simulink model "ASM_Traffic_new"  (R2024a)
settings: Solver=ode1  StartTime=SIM.tstart.v  StopTime=SIM.tend.v  FixedStep=SIM.StepSize.v  RelTol=1e-3
PostLoadFcn:
  | if any(exist('dsrtsu_mdlpostloadfcn', 'file') ~= 0), dsrtsu_mdlpostloadfcn('Execute', bdroot); end
  | try, asm_mdl_postloadfcn(bdroot, 'UpdateModel', 3600); catch, disp(lasterr); end,
InitFcn:
  | , if any(exist('rtifpga_mdlclblib', 'file') ~= 0), rtifpga_mdlclblib('Init', bdroot); end,
  | , if any(exist('dsmpb_private', 'file') ~= 0), dsmpb_private('dsmpb_mdlclblib', 'Init', bdroot); end,
undefined symbols (not defined in the file): _to_, a0b2, ASM_BrakeHydraulics_DemoSystems, ASM_VehicleDynamics_DemoSystems, b98103fe8ad365046cd0, BrakeCircuit, CPT, Crankshaft, DiscIntNeverNeededParam, dsmsi, FinalDriveAssembly, MDL, ModeSignals, Pos_BrakePedal_Maneuver, rad, RefSignals, s_to_rpm, SIM, SoftECU, Suspension, Tire, Transmission
libraries: ASM_Traffic_lib x135, simulink x100, ASM_Utils_lib x77, ASM_VehicleDynamics_lib x70, ASM_Environment_lib x22, dsmpblib x20, dsmsilib x15, MDLD_Utils_lib x10, ASM_BrakeHydraulics_lib x3
(part 3 of 63)

== system ASM_Traffic_new/AnimationInterface/Vehicle_Lights ==
  VehicleDynamics_Animation : Inport
  Environment_Animation : Inport  Port=2
  Bus Selector : BusSelector  OutputSignals=Sw_ManualControl_Lights[1Maneuver|2Manual],Sw_BrakeLight[0Off|1On],Sw_TurnLights[0Off|1Left|2Right|3Both],ASM_Vehicle_TurnLights[]
  Bus Selector13 : BusSelector  OutputSignals=p_Brake[FL;FR;RL;RR][bar]
  Cmp_BrakePres : simulink/Logic and Bit Operations/Compare To Constant  relop=>  const=3  OutDataTypeStr=boolean
  Coding : Subsystem
  Compare_Hazard : simulink/Logic and Bit Operations/Compare To Constant  relop===  const=3  OutDataTypeStr=boolean
  Compare_Turnlight_L : simulink/Logic and Bit Operations/Compare To Constant  relop===  const=1.0  OutDataTypeStr=boolean
  Compare_Turnlight_R : simulink/Logic and Bit Operations/Compare To Constant  relop===  const=2  OutDataTypeStr=boolean
  Data Type Conversion1 : DataTypeConversion  OutDataTypeStr=boolean  SaturateOnIntegerOverflow=off  RndMeth=Floor
  Data Type Conversion2 : DataTypeConversion  OutDataTypeStr=uint32  SaturateOnIntegerOverflow=off  RndMeth=Floor
  Data Type Conversion3 : DataTypeConversion  OutDataTypeStr=uint32  SaturateOnIntegerOverflow=off  RndMeth=Floor
  Data Type Conversion4 : DataTypeConversion  OutDataTypeStr=uint32  SaturateOnIntegerOverflow=off  RndMeth=Floor
  Gain : Gain  Gain=1/4
  Multiport Switch : MultiPortSwitch  Inputs=2  SaturateOnIntegerOverflow=off  InputSameDT=off
  Multiport Switch4 : MultiPortSwitch  Inputs=2  SaturateOnIntegerOverflow=off  InputSameDT=off
  Mux : Mux  Inputs=3
  OR : Logic  Operator=OR  IconShape=distinctive  AllPortsSameDT=off  OutDataTypeStr=boolean
  OR1 : Logic  Operator=OR  IconShape=distinctive  AllPortsSameDT=off  OutDataTypeStr=boolean
  Sum of Elements : Sum  Inputs=+
  ASM_Vehicle_Lights : Outport  VectorParamsAs1DForOutWhenUnconnected=off
  wires:
  Bus Selector13/1 -> Sum of Elements/1  "<p_Brake[FL;FR;RL;RR][bar]>"
  Compare_Turnlight_L/1 -> OR/1
  Gain/1 -> Cmp_BrakePres/1
  Multiport Switch/1 -> Mux/1
  Data Type Conversion3/1 -> Multiport Switch/1, Multiport Switch4/1
  Compare_Hazard/1 -> OR/2, OR1/2
  Bus Selector/1 -> Data Type Conversion3/1  "<Sw_ManualControl_Lights[1Maneuver|2Manual]>"
  Bus Selector/3 -> Data Type Conversion2/1  "<Sw_TurnLights[0Off|1Left|2Right|3Both]>"
  Data Type Conversion4/1 -> Multiport Switch4/2
  Sum of Elements/1 -> Gain/1
  Bus Selector/4 -> Data Type Conversion4/1  "<ASM_Vehicle_TurnLights[]>"
  Bus Selector/2 -> Data Type Conversion1/1  "<Sw_BrakeLight[0Off|1On]>"
  Compare_Turnlight_R/1 -> OR1/1
  OR1/1 -> Mux/3
  Cmp_BrakePres/1 -> Multiport Switch/2
  Data Type Conversion2/1 -> Multiport Switch4/3
  OR/1 -> Mux/2
  Data Type Conversion1/1 -> Multiport Switch/3
  Multiport Switch4/1 -> Compare_Hazard/1, Compare_Turnlight_R/1, Compare_Turnlight_L/1
  Mux/1 -> Coding/1(In)
  Coding/1(Out) -> ASM_Vehicle_Lights/1
  Environment_Animation/1 -> Bus Selector/1
  VehicleDynamics_Animation/1 -> Bus Selector13/1

== system ASM_Traffic_new/DomainControl/DriverAssistance ==
  note: Driver Assistance
  In : Inport
  Control : Subsystem
  Interface_In : Subsystem
  Interface_Out : Subsystem
  SignalInterface : Subsystem
  Out : Outport  VectorParamsAs1DForOutWhenUnconnected=off
  wires:
  In/1 -> Interface_In/1(In)
  Interface_In/1(Out) -> SignalInterface/1(In), Control/1(Interface_In)
  Interface_Out/1(Out) -> Out/1
  Control/1(Control) -> Interface_Out/1(In)

== system ASM_Traffic_new/DomainControl/StartSystem ==
  note: Start System
  In : Inport
  Control : Subsystem
  Interface_In : Subsystem
  Interface_Out : Subsystem
  SignalInterface : Subsystem
  Out : Outport  VectorParamsAs1DForOutWhenUnconnected=off
  wires:
  In/1 -> Interface_In/1(In)
  Interface_In/1(Out) -> SignalInterface/1(In), Control/1(Interface_In)
  Interface_Out/1(Out) -> Out/1
  Control/1(Control) -> Interface_Out/1(In)

== system ASM_Traffic_new/DomainControl/TorqueManager ==
  note: Torque Manager Basic
  In : Inport
  Control : Subsystem
  Interface_In : Subsystem
  Interface_Out : Subsystem
  SignalInterface : Subsystem
  Out : Outport  VectorParamsAs1DForOutWhenUnconnected=off
  wires:
  In/1 -> Interface_In/1(In)
  Control/1(Control) -> Interface_Out/1(In)
  Interface_In/1(Out) -> SignalInterface/1(In), Control/1(Interface_In)
  Interface_Out/1(Out) -> Out/1

== system ASM_Traffic_new/Driver/Interface_In ==
  note: Driver
  In : Inport
  Bus Creator1 : BusCreator  Inputs=1
  Bus Selector4 : BusSelector  OutputSignals=Environment.Plant.Sw_ModelPortBlocks[0Disabled|1Enabled],Environment.Plant.Sw_ModelDeskPlottingInterface[0Disabled|1Enabled],VehicleDynamics.Plant.v_x_Vehicle_CoG[km|h],VehicleDynamics.Plant.v_y_Vehicle_CoG[km|h],VehicleDynamics.Plant.Pos_x_Vehicle_CoorSys_E[m],VehicleDynamics.Plant.Pos_y_Vehicle_CoorSys_E[m],VehicleDynamics.Plant.Angle_Yaw_Vehicle_CoorSys_E[deg],VehicleDynamics.Plant.YawRate_Vehicle_CoG[deg|s],VehicleDynamics.Plant.m_TotalVehicle[kg],VehicleDynamics.Plant.F_Driving_Res[N],VehicleDynamics.Plant.Pos_x_CoG_Vehicle_Total[m],VehicleDynamics.Plant.Inertia_z_Vehicle_Total[kgm2],VehicleDynamics.Plant.CorneringStiffness_Tire_Front[N|rad],VehicleDynamics.Plant.CorneringStiffness_Tire_Rear[N|rad],VehicleDynamics.Plant.i_Steering_Mean[],Drivetrain.Plant.n_Engine[rpm],Drivetrain.Plant.omega_Out_Trm[rad|s],DomainControl.TorqueManager.Control.State_Engine[0|1|2|3|4],Environment.Plant.Reset_States[0|1],Environment.Plant.s_Vehicle_Init[m],Environment.Plant.Route_Direction_Init[],Environment.Plant.s_Total_Vehicle_Road[m],Environment.Plant.Curv_Preview_Road[1|m],Environment.Plant.Speed_Limit_Preview_Road[km|h],Environment.Plant.Pos_z_Preview_Road[m],Environment.Plant.Roll_Preview_Road[deg],Environment.Plant.Pitch_Preview_Road[deg],Environment.Plant.x_Preview_DriverCurv[m],Environment.Plant.y_Preview_DriverCurv[m],Environment.Plant.Pos_x_Preview_Road[m],Environment.Plant.Pos_y_Preview_Road[m],Environment.Plant.Dist_Border_Left[m],Environment.Plant.Dist_Border_Right[m],Environment.Plant.Curv_Vehicle_Road[1|m],Environment.Plant.Angle_Yaw_Veh_Road[deg],Environment.Plant.Pos_AccPedal_Maneuver[%],Environment.Plant.Pos_BrakePedal_Maneuver[%],Environment.Plant.Pos_ClutchPedal_Maneuver[%],Environment.Plant.Gear_Maneuver[],Environment.Plant.Angle_SteeringWheel_Maneuver[deg],Environment.Plant.SelectorLever_Maneuver[-3T|-2P|-1R|0N|1D],Environment.Plant.v_Vehicle_Ref_Maneuver[m|s],Environment.Plant.v_Vehicle_Preview_Ref_Maneuver[m|s],Environment.Plant.a_x_Max[m|s2],Environment.Plant.a_x_Min[m|s2],Environment.Plant.a_y_Max[m|s2],Environment.Plant.Gear_Max[0Off|1_n],Environment.Plant.a_x_Vehicle_Ref_TrafficDriver[m|s2],Environment.Plant.Width_Deadzone_LatCtrl[m],Environment.Plant.Pos_x_Ref_Vehicle_Road[m],Environment.Plant.Pos_y_Ref_Vehicle_Road[m],Environment.Plant.Enable_v_Init[0|1],Drivetrain.Plant.Mode_Transmission[1Manual|2Automatic],Environment.Plant.Mode_AcceleratorBrake[1Stim|2Driver],Environment.Plant.Mode_GearClutch[1Stim|2Driver|3OpenClutch|4RefGear],Environment.Plant.Mode_Steer[1Stim|2Driver|3Fix],Environment.Plant.Sw_LatDriver[1LatCtrl1|2LatCtrl2],Environment.Plant.Mode_LatCtrl[1Pos|2Yaw],Environment.Plant.Mode_AdaptVelocityToRoad[1Off|2On],Environment.Plant.Mode_ForceToRoad[1Off|2On],Environment.Plant.Mode_SelectorLever[1Stim|2Driver],Environment.Plant.Mode_CurvatureCalculation[1Road|2Driver],Environment.Plant.Mode_TrafficDriver[1Off|2On],Engine.Control.State_StartStop[1Off|2NotReady|3Ready|4EngStopped],Engine.Control.n_Engine_Idle_Set[rpm],Environment.Plant.Lane_ID_Vehicle[]
  ModelSignals : Subsystem
  Out : Outport  VectorParamsAs1DForOutWhenUnconnected=off
  wires:
  Bus Selector4/2 -> ModelSignals/2(Sw_ModelDeskPlottingInterface[0Disabled|1Enabled])  "<Sw_ModelDeskPlottingInterface[0Disabled|1Enabled]>"
  Bus Selector4/1 -> ModelSignals/1(Sw_ModelPortBlocks[0Disabled|1Enabled])  "<Sw_ModelPortBlocks[0Disabled|1Enabled]>"
  In/1 -> Bus Selector4/1
  Bus Selector4/51 -> ModelSignals/51(Pos_y_Ref_Vehicle_Road[m])  "<Pos_y_Ref_Vehicle_Road[m]>"
  Bus Selector4/50 -> ModelSignals/50(Pos_x_Ref_Vehicle_Road[m])  "<Pos_x_Ref_Vehicle_Road[m]>"
  Bus Selector4/49 -> ModelSignals/49(Width_Deadzone_LatCtrl[m])  "<Width_Deadzone_LatCtrl[m]>"
  Bus Selector4/48 -> ModelSignals/48(a_x_Vehicle_Ref_TrafficDriver[m|s2])  "<a_x_Vehicle_Ref_TrafficDriver[m|s2]>"
  Bus Selector4/47 -> ModelSignals/47(Gear_Max[0Off|1_n])  "<Gear_Max[0Off|1_n]>"
  Bus Selector4/46 -> ModelSignals/46(a_y_Max[m|s2])  "<a_y_Max[m|s2]>"
  Bus Selector4/45 -> ModelSignals/45(a_x_Min[m|s2])  "<a_x_Min[m|s2]>"
  Bus Selector4/44 -> ModelSignals/44(a_x_Max[m|s2])  "<a_x_Max[m|s2]>"
  Bus Selector4/43 -> ModelSignals/43(v_Vehicle_Preview_Ref_Maneuver[m|s])  "<v_Vehicle_Preview_Ref_Maneuver[m|s]>"
  Bus Selector4/42 -> ModelSignals/42(v_Vehicle_Ref_Maneuver[m|s])  "<v_Vehicle_Ref_Maneuver[m|s]>"
  Bus Selector4/41 -> ModelSignals/41(SelectorLever_Maneuver[-3T|-2P|-1R|0N|1D])  "<SelectorLever_Maneuver[-3T|-2P|-1R|0N|1D]>"
  Bus Selector4/40 -> ModelSignals/40(Angle_SteeringWheel_Maneuver[deg])  "<Angle_SteeringWheel_Maneuver[deg]>"
  Bus Selector4/39 -> ModelSignals/39(Gear_Maneuver[])  "<Gear_Maneuver[]>"
  Bus Selector4/38 -> ModelSignals/38(Pos_ClutchPedal_Maneuver[%])  "<Pos_ClutchPedal_Maneuver[%]>"
  Bus Selector4/37 -> ModelSignals/37(Pos_BrakePedal_Maneuver[%])  "<Pos_BrakePedal_Maneuver[%]>"
  Bus Selector4/36 -> ModelSignals/36(Pos_AccPedal_Maneuver[%])  "<Pos_AccPedal_Maneuver[%]>"
  Bus Selector4/35 -> ModelSignals/35(Angle_Yaw_Veh_Road[deg])  "<Angle_Yaw_Veh_Road[deg]>"
  Bus Selector4/34 -> ModelSignals/34(Curv_Veh_Road[1|m])  "<Curv_Vehicle_Road[1|m]>"
  Bus Selector4/33 -> ModelSignals/33(Dist_Border_Right[m])  "<Dist_Border_Right[m]>"
  Bus Selector4/32 -> ModelSignals/32(Dist_Border_Left[m])  "<Dist_Border_Left[m]>"
  Bus Selector4/31 -> ModelSignals/31(Pos_y_Preview_Road[m])  "<Pos_y_Preview_Road[m]>"
  Bus Selector4/30 -> ModelSignals/30(Pos_x_Preview_Road[m])  "<Pos_x_Preview_Road[m]>"
  Bus Selector4/29 -> ModelSignals/29(Pos_y_Preview_DriverCurv[m])  "<y_Preview_DriverCurv[m]>"
  Bus Selector4/28 -> ModelSignals/28(Pos_x_Preview_DriverCurv[m])  "<x_Preview_DriverCurv[m]>"
  Bus Selector4/27 -> ModelSignals/27(Pitch_Preview_Road[deg])  "<Pitch_Preview_Road[deg]>"
  Bus Selector4/26 -> ModelSignals/26(Roll_Preview_Road[deg])  "<Roll_Preview_Road[deg]>"
  Bus Selector4/25 -> ModelSignals/25(Pos_z_Preview_Road[m])  "<Pos_z_Preview_Road[m]>"
  Bus Selector4/24 -> ModelSignals/24(Speed_Limit_Preview_Road[km|h])  "<Speed_Limit_Preview_Road[km|h]>"
  Bus Selector4/23 -> ModelSignals/23(Curv_Preview_Road[1|m])  "<Curv_Preview_Road[1|m]>"
  Bus Selector4/22 -> ModelSignals/22(s_Total_Vehicle_Road[m])  "<s_Total_Vehicle_Road[m]>"
  Bus Selector4/21 -> ModelSignals/21(Route_Direction_Init[])  "<Route_Direction_Init[]>"
  Bus Selector4/20 -> ModelSignals/20(s_Vehicle_Init[m])  "<s_Vehicle_Init[m]>"
  Bus Selector4/19 -> ModelSignals/19(Reset_States[0|1])  "<Reset_States[0|1]>"
  Bus Creator1/1 -> Out/1
  Bus Selector4/52 -> ModelSignals/52(Enable_v_Init[0|1])  "<Enable_v_Init[0|1]>"
  Bus Selector4/53 -> ModelSignals/53(Mode_Transmission[1Manual|2Automatic])  "<Mode_Transmission[1Manual|2Automatic]>"
  Bus Selector4/54 -> ModelSignals/54(Mode_AcceleratorBrake[1Stim|2Driver])  "<Mode_AcceleratorBrake[1Stim|2Driver]>"
  Bus Selector4/55 -> ModelSignals/55(Mode_GearClutch[1Stim|2Driver|3OpenClutch|4RefGear])  "<Mode_GearClutch[1Stim|2Driver|3OpenClutch|4RefGear]>"
  Bus Selector4/56 -> ModelSignals/56(Mode_Steer[1Stim|2Driver|3Fix])  "<Mode_Steer[1Stim|2Driver|3Fix]>"
  Bus Selector4/57 -> ModelSignals/57(Sw_LatDriver[1LatCtrl1|2LatCtrl2])  "<Sw_LatDriver[1LatCtrl1|2LatCtrl2]>"
  Bus Selector4/58 -> ModelSignals/58(Mode_LatCtrl[1Pos|2Yaw])  "<Mode_LatCtrl[1Pos|2Yaw]>"
  Bus Selector4/59 -> ModelSignals/59(Mode_AdaptVelocityToRoad[1Off|2On])  "<Mode_AdaptVelocityToRoad[1Off|2On]>"
  Bus Selector4/60 -> ModelSignals/60(Mode_ForceToRoad[1Off|2On])  "<Mode_ForceToRoad[1Off|2On]>"
  Bus Selector4/61 -> ModelSignals/61(Mode_SelectorLever[1Stim|2Driver])  "<Mode_SelectorLever[1Stim|2Driver]>"
  Bus Selector4/62 -> ModelSignals/62(Mode_CurvatureCalculation[1Road|2Driver])  "<Mode_CurvatureCalculation[1Road|2Driver]>"
  Bus Selector4/63 -> ModelSignals/63(Mode_TrafficDriver[1Off|2On])  "<Mode_TrafficDriver[1Off|2On]>"
  Bus Selector4/65 -> ModelSignals/65(n_Engine_Idle_Set[rpm])  "<n_Engine_Idle_Set[rpm]>"
  Bus Selector4/64 -> ModelSignals/64(State_StartStop[1Off|2NotReady|3Ready|4EngStopped])  "<State_StartStop[1Off|2NotReady|3Ready|4EngStopped]>"
  Bus Selector4/18 -> ModelSignals/18(State_Engine[0|1|2|3|4])  "<State_Engine[0|1|2|3|4]>"
  Bus Selector4/17 -> ModelSignals/17(omega_Out_Trm[rad|s])  "<omega_Out_Trm[rad|s]>"
  Bus Selector4/16 -> ModelSignals/16(n_Engine[rpm])  "<n_Engine[rpm]>"
  Bus Selector4/15 -> ModelSignals/15(i_Steering_Mean[])  "<i_Steering_Mean[]>"
  Bus Selector4/14 -> ModelSignals/14(CorneringStiffness_Tire_Rear[N|rad])  "<CorneringStiffness_Tire_Rear[N|rad]>"
  Bus Selector4/13 -> ModelSignals/13(CorneringStiffness_Tire_Front[N|rad])  "<CorneringStiffness_Tire_Front[N|rad]>"
  Bus Selector4/12 -> ModelSignals/12(Inertia_z_Vehicle_Total[kgm2])  "<Inertia_z_Vehicle_Total[kgm2]>"
  Bus Selector4/11 -> ModelSignals/11(Pos_x_CoG_Vehicle_Total[m])  "<Pos_x_CoG_Vehicle_Total[m]>"
  Bus Selector4/10 -> ModelSignals/10(F_Driving_Res[N])  "<F_Driving_Res[N]>"
  Bus Selector4/9 -> ModelSignals/9(m_Total_Vehicle[kg])  "<m_TotalVehicle[kg]>"
  Bus Selector4/8 -> ModelSignals/8(YawRate_Vehicle[deg|s])  "<YawRate_Vehicle_CoG[deg|s]>"
  Bus Selector4/7 -> ModelSignals/7(Angle_Yaw_Vehicle_CoorSys_E[deg])  "<Angle_Yaw_Vehicle_CoorSys_E[deg]>"
  Bus Selector4/6 -> ModelSignals/6(Pos_y_Vehicle_CoorSys_E[m])  "<Pos_y_Vehicle_CoorSys_E[m]>"
  Bus Selector4/5 -> ModelSignals/5(Pos_x_Vehicle_CoorSys_E[m])  "<Pos_x_Vehicle_CoorSys_E[m]>"
  Bus Selector4/4 -> ModelSignals/4(v_y_Vehicle_CoG[km|h])  "<v_y_Vehicle_CoG[km|h]>"
  Bus Selector4/3 -> ModelSignals/3(v_x_Vehicle_CoG[km|h])  "<v_x_Vehicle_CoG[km|h]>"
  ModelSignals/1(Out) -> Bus Creator1/1
  Bus Selector4/66 -> ModelSignals/66(Lane_ID_Vehicle[])  "<Lane_ID_Vehicle[]>"

== system ASM_Traffic_new/Driver/Interface_Out ==
  note: Driver
  In : Inport
  Bus Creator1 : BusCreator  Inputs=1
  Bus Selector2 : BusSelector  OutputSignals=OutputSignals.Pos_AccPedal[%],OutputSignals.Pos_BrakePedal[%],OutputSignals.Pos_ClutchPedal[%],OutputSignals.Gear[],OutputSignals.SelectorLever[-3T|-2P|-1R|0N|1D],OutputSignals.s_Preview[m],OutputSignals.Angle_SteeringWheel[deg],LongitudinalController.LongCtrl.t_Preview[s]
  Plant_ModelSignals : Subsystem
  Out : Outport  VectorParamsAs1DForOutWhenUnconnected=off
  wires:
  Bus Selector2/6 -> Plant_ModelSignals/6(s_Preview[m])  "<s_Preview[m]>"
  Bus Selector2/8 -> Plant_ModelSignals/8(t_Preview_vRef_Driver[s])  "<t_Preview[s]>"
  Bus Selector2/5 -> Plant_ModelSignals/5(SelectorLever[-3T|-2P|-1R|0N|1D])  "<SelectorLever[-3T|-2P|-1R|0N|1D]>"
  Bus Selector2/4 -> Plant_ModelSignals/4(Gear[])  "<Gear[]>"
  Bus Selector2/3 -> Plant_ModelSignals/3(Pos_ClutchPedal[%])  "<Pos_ClutchPedal[%]>"
  Bus Selector2/2 -> Plant_ModelSignals/2(Pos_BrakePedal[%])  "<Pos_BrakePedal[%]>"
  Bus Selector2/1 -> Plant_ModelSignals/1(Pos_AccPedal[%])  "<Pos_AccPedal[%]>"
  In/1 -> Bus Selector2/1
  Bus Selector2/7 -> Plant_ModelSignals/7(Angle_SteeringWheel[deg])  "<Angle_SteeringWheel[deg]>"
  Bus Creator1/1 -> Out/1  "Driver"
  Plant_ModelSignals/1(Out) -> Bus Creator1/1

== system ASM_Traffic_new/Driver/Plant ==
  note: Driver
  Interface_In : Inport
  Driver : Subsystem
  UserInterface : Subsystem
  Plant : Outport  VectorParamsAs1DForOutWhenUnconnected=off
  wires:
  Driver/1(ASMSignalBus) -> Plant/1, UserInterface/1(In)
  Interface_In/1 -> Driver/2(Interface_In), UserInterface/2(Interface_In)
  UserInterface/1(Out) -> Driver/1(UserInterface)

== system ASM_Traffic_new/Driver/SignalInterface ==
  In : Inport
  ASMSignalInterface : Subsystem  mask(ASM_SIGNAL_INTERFACE){LabelTextfield=Driver}
      mask prompts: LabelTextfield "Label"
      mask help:
      | The ASMSignalInterface block processes the ASMSignalBus and provides a vector-based interface for each signal (e.g. ModelDesk Plotting).
      |
      | Always push the update button after you have changed the signal bus structure in order to synchronize the signal interface. The update may take a few seconds.
      | A modified model must be reloaded in ModelDesk to keep consistency of ModelDesk and simulation model plot signals. Therefore select ''Update Model'' from the ''Simulation Model'' context menu of the ModelDesk Project Navigator.
      settings: AttributesFormatString=Label: %<LabelTextfield>
      settings: CopyFcn=|
      | try
      |  set_param(gcb,'LinkStatus', 'none')
      | catch
      | end
      mask Help: eval(['asm_modelhelp(gcbh,''tool'',''ASM_Utils_lib'', ''ASMSIGNALINTERFACE'')'])
      mask DialogControl Hint Prompt: For changes of Label first apply change and then push "Update".
      mask DialogControl UpdateButton Prompt: Update
      mask DialogControl UpdateButton Callback: asm_mdld_plot_block_update(bdroot(gcb), 'update', 'current');
      mask DialogControl UpdateAllButton Prompt: Update All
      mask DialogControl UpdateAllButton Callback: asm_mdld_plot_block_update(bdroot(gcb), 'update', 'all');
  Bus Selector Disable Signals : BusSelector  OutputSignals=ExternalModel.Sw_ModelPortBlocks[0Disabled|1Enabled],ExternalModel.Sw_ModelDeskPlottingInterface[0Disabled|1Enabled]
  ExternalOutports : Subsystem  TreatAsAtomicUnit=on
  wires:
  Bus Selector Disable Signals/2 -> ASMSignalInterface/Enable  "<Sw_ModelDeskPlottingInterface[0Disabled|1Enabled]>"
  Bus Selector Disable Signals/1 -> ExternalOutports/Enable  "<Sw_ModelPortBlocks[0Disabled|1Enabled]>"
  In/1 -> Bus Selector Disable Signals/1
  [ASMBUS_Driver_Plant] -> ASMSignalInterface/1(ASMSignalBus), ExternalOutports/1(In1)

== system ASM_Traffic_new/Drivetrain/Control ==
  note: Drivetrain Control
  Interface_In : Inport
  Plant : Inport  Port=2
  SoftECU_Drivetrain : Subsystem
  Sw_ECU_Signals : Subsystem
  UserInterface : Subsystem
  Control : Outport  VectorParamsAs1DForOutWhenUnconnected=off
  wires:
  Interface_In/1 -> SoftECU_Drivetrain/2(Interface_In), Sw_ECU_Signals/2(ExternalECU)
  SoftECU_Drivetrain/2(Out) -> Sw_ECU_Signals/1(SoftECU)
  Sw_ECU_Signals/1(ECU_Signals) -> Control/1
  SoftECU_Drivetrain/1(ASMSignalBus) -> UserInterface/1(In)
  UserInterface/1(Out) -> SoftECU_Drivetrain/1(UserInterface)
  Plant/1 -> SoftECU_Drivetrain/3(Plant)

== system ASM_Traffic_new/Drivetrain/Interface_In ==
  note: Drivetrain
  In : Inport
  Bus Creator1 : BusCreator  Inputs=2
  Bus Selector5 : BusSelector  OutputSignals=Environment.Plant.Sw_ModelPortBlocks[0Disabled|1Enabled],Environment.Plant.Sw_ModelDeskPlottingInterface[0Disabled|1Enabled],Environment.Plant.n_Engine_Set[rpm],Environment.Plant.Sw_Testbench[0Off|1On],Driver.Plant.Pos_ClutchPedal[%],Driver.Plant.Gear[],Environment.Plant.Reset_States[0|1],Engine.Plant.Trq_MeanEff_Engine[Nm],VehicleDynamics.Plant.omega_Wheel[FL;FR;RL;RR][rad|s],Environment.Plant.Enable_v_Init[0|1],Driver.Plant.Pos_AccPedal[%],Driver.Plant.SelectorLever[-3T|-2P|-1R|0N|1D],Environment.Plant.Sw_TipShift_Maneuver[-1Down|0Off|1Up],Environment.Plant.Gear_Maneuver[],Environment.Plant.Mode_GearClutch[1Stim|2Driver|3OpenClutch|4RefGear],Environment.Plant.Gear_Max[0Off|1_n],DomainControl.TorqueManager.Control.State_Engine[0|1|2|3|4],Engine.Control.State_StartStop[1Off|2NotReady|3Ready|4EngStopped],Engine.Control.Sw_Starter[0Off|1On],Engine.Control.CrankAngle_Cyl[aTDC],Engine.Plant.Type_Engine[0Unkown|1Other|2Otto|3Diesel|4Electric]
  Bus Selector51 : BusSelector  OutputSignals=Environment.Plant.Sw_ModelPortBlocks[0Disabled|1Enabled]
  ExternalSignals : Subsystem
  ModelSignals : Subsystem
  Out : Outport  VectorParamsAs1DForOutWhenUnconnected=off
  wires:
  Bus Selector51/1 -> ExternalSignals/Enable  "<Sw_ModelPortBlocks[0Disabled|1Enabled]>"
  ExternalSignals/1(ExternalECU_Transmission_Out) -> Bus Creator1/2
  Bus Selector5/2 -> ModelSignals/2(Sw_ModelDeskPlottingInterface[0Disabled|1Enabled])  "<Sw_ModelDeskPlottingInterface[0Disabled|1Enabled]>"
  Bus Selector5/1 -> ModelSignals/1(Sw_ModelPortBlocks[0Disabled|1Enabled])  "<Sw_ModelPortBlocks[0Disabled|1Enabled]>"
  In/1 -> Bus Selector51/1, Bus Selector5/1
  Bus Creator1/1 -> Out/1
  Bus Selector5/3 -> ModelSignals/3(n_Engine_Set[rpm])  "<n_Engine_Set[rpm]>"
  Bus Selector5/4 -> ModelSignals/4(Sw_Testbench[0Off|1On])  "<Sw_Testbench[0Off|1On]>"
  Bus Selector5/5 -> ModelSignals/5(Pos_ClutchPedal[%])  "<Pos_ClutchPedal[%]>"
  Bus Selector5/6 -> ModelSignals/6(Gear[])  "<Gear[]>"
  Bus Selector5/7 -> ModelSignals/7(Reset_States[0|1])  "<Reset_States[0|1]>"
  Bus Selector5/9 -> ModelSignals/9(omega_Wheel[FL;FR;RL;RR][rad|s])  "<omega_Wheel[FL;FR;RL;RR][rad|s]>"
  Bus Selector5/8 -> ModelSignals/8(Trq_MeanEff_Engine[Nm])  "<Trq_MeanEff_Engine[Nm]>"
  Bus Selector5/10 -> ModelSignals/10(Enable_v_Init[0|1])  "<Enable_v_Init[0|1]>"
  Bus Selector5/11 -> ModelSignals/11(Pos_AccPedal[%])  "<Pos_AccPedal[%]>"
  Bus Selector5/12 -> ModelSignals/12(SelectorLever[-3T|-2P|-1R|0N|1D])  "<SelectorLever[-3T|-2P|-1R|0N|1D]>"
  Bus Selector5/13 -> ModelSignals/13(Sw_TipShift[-1Down|0Off|1Up])  "<Sw_TipShift_Maneuver[-1Down|0Off|1Up]>"
  Bus Selector5/14 -> ModelSignals/14(Gear_Maneuver[])  "<Gear_Maneuver[]>"
  Bus Selector5/15 -> ModelSignals/15(Mode_GearClutch[1Stim|2Driver|3OpenClutch|4RefGear])  "<Mode_GearClutch[1Stim|2Driver|3OpenClutch|4RefGear]>"
  Bus Selector5/16 -> ModelSignals/16(Gear_Max[0Off|1_n])  "<Gear_Max[0Off|1_n]>"
  Bus Selector5/17 -> ModelSignals/17(State_Engine[0|1|2|3|4])  "<State_Engine[0|1|2|3|4]>"
  Bus Selector5/18 -> ModelSignals/18(State_StartStop[1Off|2NotReady|3Ready|4EngStopped])  "<State_StartStop[1Off|2NotReady|3Ready|4EngStopped]>"
  Bus Selector5/19 -> ModelSignals/19(Sw_Starter[0|1])  "<Sw_Starter[0Off|1On]>"
  Bus Selector5/20 -> ModelSignals/20(CrankAngle_Cyl[aTDC])  "<CrankAngle_Cyl[aTDC]>"
  ModelSignals/1(Out) -> Bus Creator1/1
  Bus Selector5/21 -> ModelSignals/21(Type_Engine_1[0Unkown|1Other|2Otto|3Diesel|4Electric])  "<Type_Engine[0Unkown|1Other|2Otto|3Diesel|4Electric]>"

== system ASM_Traffic_new/Drivetrain/Interface_Out ==
  note: Drivetrain
  In : Inport
  Animation : Subsystem
  Bus Creator1 : BusCreator  Inputs=3
  Bus Selector2 : BusSelector  OutputSignals=Plant.Drivetrain.Crankshaft.n_Engine[rpm],Plant.Drivetrain.Transmission.OutputSignals.omega_Out_Trm[rad|s],Plant.Drivetrain.Transmission.OutputSignals.Gear[],Plant.Drivetrain.FinalDriveAssembly.i_FinalDrive[],Plant.Drivetrain.FinalDriveAssembly.i_FrontDrive[],Plant.Drivetrain.FinalDriveAssembly.i_RearDrive[],Plant.Drivetrain.FinalDriveAssembly.TrqDistri_Front_Rear[0_1],Plant.Drivetrain.FinalDriveAssembly.Trq_Out_Front_Diff[Nm],Plant.Drivetrain.FinalDriveAssembly.Trq_Shaft[FL;FR;RL;RR][Nm],Plant.Drivetrain.Transmission.OutputSignals.i_unsync_Trm[],Plant.UserInterface.Sw_CrankShaft_Reset[0Disabled|1Enabled],Plant.UserInterface.Mode_Transmission[1Manual|2Automatic],Plant.UserInterface.Mode_Drivetrain[1AWD|2FWD|3RWD|4FF-4WD|5FF],Plant.Drivetrain.Type_Engine_1[0Unkown|1Other|2Otto|3Diesel|4Electric],Plant.Drivetrain.Trq_MeanEff_Engine[Nm],Plant.Drivetrain.Crankshaft.n_Engine[rpm]
  Bus Selector3 : BusSelector  OutputSignals=Plant.Drivetrain.Crankshaft.n_Engine[rpm],Plant.Drivetrain.Transmission.OutputSignals.Gear[]
  Bus Selector4 : BusSelector  OutputSignals=Control.Factor_Trq_Engine_Red[%],Control.Ctrl_Parking_Pawl[0|1]
  Control_ModelSignals : Subsystem
  Plant_ModelSignals : Subsystem
  Trq_BSG[Nm] : Constant  Value=0
  Trq_Engine_2[Nm] : Constant  Value=0
  Type_Engine_2[0Unkown|1Other|2Otto|3Diesel|4Electric] : Constant  Value=0
  n_Engine_2[rpm] : Constant  Value=0
  Out : Outport  VectorParamsAs1DForOutWhenUnconnected=off
  wires:
  n_Engine_2[rpm]/1 -> Plant_ModelSignals/19(n_Engine_2[rpm])
  Bus Selector2/16 -> Plant_ModelSignals/16(n_Engine_1[rpm])  "<n_Engine[rpm]>"
  Bus Selector2/9 -> Plant_ModelSignals/9(Trq_Shaft[FL;FR;RL;RR][Nm])  "<Trq_Shaft[FL;FR;RL;RR][Nm]>"
  Bus Selector2/8 -> Plant_ModelSignals/8(Trq_Out_Front_Diff[Nm])  "<Trq_Out_Front_Diff[Nm]>"
  Bus Selector2/7 -> Plant_ModelSignals/7(TrqDistri_Front_Rear[0_1])  "<TrqDistri_Front_Rear[0_1]>"
  Bus Selector2/6 -> Plant_ModelSignals/6(i_RearDrive[])  "<i_RearDrive[]>"
  Bus Selector2/5 -> Plant_ModelSignals/5(i_FrontDrive[])  "<i_FrontDrive[]>"
  Bus Selector2/2 -> Plant_ModelSignals/2(omega_Out_Trm[rad|s])  "<omega_Out_Trm[rad|s]>"
  Bus Selector3/2 -> Animation/2(Gear[])  "<Gear[]>"
  Bus Selector3/1 -> Animation/1(n_Engine[rpm])  "<n_Engine[rpm]>"
  Bus Selector2/3 -> Plant_ModelSignals/3(Gear[])  "<Gear[]>"
  Bus Selector2/1 -> Plant_ModelSignals/1(n_Engine[rpm])  "<n_Engine[rpm]>"
  Bus Selector2/4 -> Plant_ModelSignals/4(i_FinalDrive[])  "<i_FinalDrive[]>"
  Bus Selector2/10 -> Plant_ModelSignals/10(i_unsync_Trm[])  "<i_unsync_Trm[]>"
  Bus Creator1/1 -> Out/1  "Drivetrain"
  Bus Selector4/2 -> Control_ModelSignals/2(Ctrl_Parking_Pawl[0|1])  "<Ctrl_Parking_Pawl[0|1]>"
  In/1 -> Bus Selector3/1, Bus Selector2/1, Bus Selector4/1
  Bus Selector4/1 -> Control_ModelSignals/1(Factor_Trq_Engine_Red[%])  "<Factor_Trq_Engine_Red[%]>"
  Control_ModelSignals/1(Out) -> Bus Creator1/1
  Trq_BSG[Nm]/1 -> Plant_ModelSignals/20(Trq_BSG[Nm])
  Bus Selector2/11 -> Plant_ModelSignals/11(Sw_CrankShaft_Reset[0Disabled|1Enabled])  "<Sw_CrankShaft_Reset[0Disabled|1Enabled]>"
  Bus Selector2/12 -> Plant_ModelSignals/12(Mode_Transmission[1Manual|2Automatic])  "<Mode_Transmission[1Manual|2Automatic]>"
  Bus Selector2/13 -> Plant_ModelSignals/13(Mode_Drivetrain[1|2|3|4|5])  "<Mode_Drivetrain[1AWD|2FWD|3RWD|4FF-4WD|5FF]>"
  Plant_ModelSignals/1(Out) -> Bus Creator1/2
  Animation/1(Out) -> Bus Creator1/3
  Bus Selector2/14 -> Plant_ModelSignals/14(Type_Engine_1[0Unkown|1Other|2Otto|3Diesel|4Electric])  "<Type_Engine_1[0Unkown|1Other|2Otto|3Diesel|4Electric]>"
  Type_Engine_2[0Unkown|1Other|2Otto|3Diesel|4Electric]/1 -> Plant_ModelSignals/17(Type_Engine_2[0Unkown|1Other|2Otto|3Diesel|4Electric])
  Bus Selector2/15 -> Plant_ModelSignals/15(Trq_Engine_1[Nm])  "<Trq_MeanEff_Engine[Nm]>"
  Trq_Engine_2[Nm]/1 -> Plant_ModelSignals/18(Trq_Engine_2[Nm])

== system ASM_Traffic_new/Drivetrain/Plant ==
  note: Drivetrain
  Interface_In : Inport
  Control : Inport  Port=2
  Bus Creator : BusCreator  Inputs=2
  Drivetrain : Subsystem
  UserInterface : Subsystem
  Plant : Outport  VectorParamsAs1DForOutWhenUnconnected=off
  wires:
  Interface_In/1 -> Drivetrain/2(Interface_In)
  Control/1 -> Drivetrain/3(Control)
  UserInterface/1(Out) -> Drivetrain/1(UserInterface), Bus Creator/2
  Drivetrain/1(ASMSignalBus) -> UserInterface/1(In), Bus Creator/1
  Bus Creator/1 -> Plant/1  "Plant"

== system ASM_Traffic_new/Drivetrain/SignalInterface ==
  In : Inport
  ASMSignalInterface : Subsystem  mask(ASM_SIGNAL_INTERFACE){LabelTextfield=Drivetrain}
      mask prompts: LabelTextfield "Label"
      mask help:
      | The ASMSignalInterface block processes the ASMSignalBus and provides a vector-based interface for each signal (e.g. ModelDesk Plotting).
      |
      | Always push the update button after you have changed the signal bus structure in order to synchronize the signal interface. The update may take a few seconds.
      | A modified model must be reloaded in ModelDesk to keep consistency of ModelDesk and simulation model plot signals. Therefore select ''Update Model'' from the ''Simulation Model'' context menu of the ModelDesk Project Navigator.
      settings: AttributesFormatString=Label: %<LabelTextfield>
      settings: CopyFcn=|
      | try
      |  set_param(gcb,'LinkStatus', 'none')
      | catch
      | end
      mask Help: eval(['asm_modelhelp(gcbh,''tool'',''ASM_Utils_lib'', ''ASMSIGNALINTERFACE'')'])
      mask DialogControl Hint Prompt: For changes of Label first apply change and then push "Update".
      mask DialogControl UpdateButton Prompt: Update
      mask DialogControl UpdateButton Callback: asm_mdld_plot_block_update(bdroot(gcb), 'update', 'current');
      mask DialogControl UpdateAllButton Prompt: Update All
      mask DialogControl UpdateAllButton Callback: asm_mdld_plot_block_update(bdroot(gcb), 'update', 'all');
  Bus Creator : BusCreator  Inputs=2
  Bus Selector Disable Signals : BusSelector  OutputSignals=ExternalModel.Sw_ModelPortBlocks[0Disabled|1Enabled],ExternalModel.Sw_ModelDeskPlottingInterface[0Disabled|1Enabled]
  ExternalOutports : Subsystem  TreatAsAtomicUnit=on
  wires:
  Bus Selector Disable Signals/2 -> ASMSignalInterface/Enable  "<Sw_ModelDeskPlottingInterface[0Disabled|1Enabled]>"
  Bus Selector Disable Signals/1 -> ExternalOutports/Enable  "<Sw_ModelPortBlocks[0Disabled|1Enabled]>"
  In/1 -> Bus Selector Disable Signals/1
  [ASMBUS_Drivetrain_Plant] -> Bus Creator/2, ExternalOutports/1(In1)
  [ASMBUS_Drivetrain_Control] -> Bus Creator/1
  Bus Creator/1 -> ASMSignalInterface/1(ASMSignalBus)

== system ASM_Traffic_new/ElectricalSystem/Control ==
  note: Electrical System Basic Control
  Interface_In : Inport
  Plant : Inport  Port=2
  SoftECU_ElectricalSystem : Subsystem
  UserInterface : Subsystem
  Control : Outport  VectorParamsAs1DForOutWhenUnconnected=off
  wires:
  SoftECU_ElectricalSystem/2(Out) -> Control/1
  Interface_In/1 -> SoftECU_ElectricalSystem/2(Interface_In)
  SoftECU_ElectricalSystem/1(ASMSignalBus) -> UserInterface/1(In)
  Plant/1 -> SoftECU_ElectricalSystem/3(Plant)
  UserInterface/1(Out) -> SoftECU_ElectricalSystem/1(UserInterface)

== system ASM_Traffic_new/ElectricalSystem/Interface_In ==
  note: Electrical System Basic
  In : Inport
  Bus Creator : BusCreator  Inputs=1
  Bus Selector : BusSelector  OutputSignals=Environment.Plant.Sw_ModelPortBlocks[0Disabled|1Enabled],Environment.Plant.Sw_ModelDeskPlottingInterface[0Disabled|1Enabled]
  ModelSignals : Subsystem
  Out : Outport  VectorParamsAs1DForOutWhenUnconnected=off
  wires:
  ModelSignals/1(Out) -> Bus Creator/1
  Bus Selector/2 -> ModelSignals/2(Sw_ModelDeskPlottingInterface[0Disabled|1Enabled])  "<Sw_ModelDeskPlottingInterface[0Disabled|1Enabled]>"
  Bus Selector/1 -> ModelSignals/1(Sw_ModelPortBlocks[0Disabled|1Enabled])  "<Sw_ModelPortBlocks[0Disabled|1Enabled]>"
  In/1 -> Bus Selector/1
  Bus Creator/1 -> Out/1

== system ASM_Traffic_new/ElectricalSystem/Interface_Out ==
  note: Electrical System Basic
  In : Inport
  Bus Creator1 : BusCreator  Inputs=2
  Bus Selector2 : BusSelector  OutputSignals=Control.SOC_Estimated_Max[%],Control.SOC_Estimated_Mean[%]
  Bus Selector7 : BusSelector  OutputSignals=Plant.Battery_LV.V_Bat[V],Plant.Battery_LV.SOC_Bat[%],Plant.Battery_LV.T_Bat[degC],Plant.Battery_HV.V_Bat[V],Plant.Battery_HV.T_Bat[degC],Plant.DCLink.V_DCLink[V]
  Control_ModelSignals : Subsystem
  I_DCDC_LS[A] : Constant  Value=0
  I_DCLink[A] : Constant  Value=0
  Plant_ModelSignals : Subsystem
  State_DCLink[0Off|1On] : Constant
  Sw_DCLink_Reset[0Disabled|1Enabled] : Constant  Value=0
  Out : Outport  VectorParamsAs1DForOutWhenUnconnected=off
  wires:
  I_DCDC_LS[A]/1 -> Plant_ModelSignals/8(I_DCDC_LS[A])
  I_DCLink[A]/1 -> Plant_ModelSignals/7(I_DCLink[A])
  Sw_DCLink_Reset[0Disabled|1Enabled]/1 -> Plant_ModelSignals/10(Sw_DCLink_Reset[0Disabled|1Enabled])
  Bus Selector7/1 -> Plant_ModelSignals/1(V_Bat_LV[V])  "<V_Bat[V]>"
  Bus Selector7/2 -> Plant_ModelSignals/2(SOC_Bat_LV[%])  "<SOC_Bat[%]>"
  Bus Selector7/3 -> Plant_ModelSignals/3(T_Bat_LV[degC])  "<T_Bat[degC]>"
  Bus Selector7/4 -> Plant_ModelSignals/4(V_Bat_HV[V])  "<V_Bat[V]>"
  Bus Selector7/5 -> Plant_ModelSignals/5(T_Bat_HV[degC])  "<T_Bat[degC]>"
  Bus Selector7/6 -> Plant_ModelSignals/6(V_DCLink[V])  "<V_DCLink[V]>"
  State_DCLink[0Off|1On]/1 -> Plant_ModelSignals/9(State_DCLink[0Off|1On])
  Bus Creator1/1 -> Out/1  "ElectricalSystem"
  Bus Selector2/2 -> Control_ModelSignals/2(SOC_Estimated_Mean[%])  "<SOC_Estimated_Mean[%]>"
  In/1 -> Bus Selector7/1, Bus Selector2/1
  Control_ModelSignals/1(Out) -> Bus Creator1/1
  Bus Selector2/1 -> Control_ModelSignals/1(SOC_Estimated_Max[%])  "<SOC_Estimated_Max[%]>"
  Plant_ModelSignals/1(Out) -> Bus Creator1/2

== system ASM_Traffic_new/ElectricalSystem/Plant ==
  note: Electrical System Basic
  Interface_In : Inport
  Control : Inport  Port=2
  ElectricalSystemBasic : Subsystem
  UserInterface : Subsystem
  Plant : Outport  VectorParamsAs1DForOutWhenUnconnected=off
  wires:
  ElectricalSystemBasic/1(ASMSignalBus) -> Plant/1, UserInterface/1(In)
  Interface_In/1 -> ElectricalSystemBasic/2(Interface_In)
  UserInterface/1(Out) -> ElectricalSystemBasic/1(UserInterface)
  Control/1 -> ElectricalSystemBasic/3(Control)

== system ASM_Traffic_new/ElectricalSystem/SignalInterface ==
  In : Inport
  ASMSignalInterface : Subsystem  mask(ASM_SIGNAL_INTERFACE){LabelTextfield=ElectricalSystem}
      mask prompts: LabelTextfield "Label"
      mask help:
      | The ASMSignalInterface block processes the ASMSignalBus and provides a vector-based interface for each signal (e.g. ModelDesk Plotting).
      |
      | Always push the update button after you have changed the signal bus structure in order to synchronize the signal interface. The update may take a few seconds.
      | A modified model must be reloaded in ModelDesk to keep consistency of ModelDesk and simulation model plot signals. Therefore select ''Update Model'' from the ''Simulation Model'' context menu of the ModelDesk Project Navigator.
      settings: AttributesFormatString=Label: %<LabelTextfield>
      settings: CopyFcn=|
      | try
      |  set_param(gcb,'LinkStatus', 'none')
      | catch
      | end
      mask Help: eval(['asm_modelhelp(gcbh,''tool'',''ASM_Utils_lib'', ''ASMSIGNALINTERFACE'')'])
      mask DialogControl Hint Prompt: For changes of Label first apply change and then push "Update".
      mask DialogControl UpdateButton Prompt: Update
      mask DialogControl UpdateButton Callback: asm_mdld_plot_block_update(bdroot(gcb), 'update', 'current');
      mask DialogControl UpdateAllButton Prompt: Update All
      mask DialogControl UpdateAllButton Callback: asm_mdld_plot_block_update(bdroot(gcb), 'update', 'all');
  Bus Selector Disable Signals : BusSelector  OutputSignals=ExternalModel.Sw_ModelDeskPlottingInterface[0Disabled|1Enabled]
  wires:
  Bus Selector Disable Signals/1 -> ASMSignalInterface/Enable  "<Sw_ModelDeskPlottingInterface[0Disabled|1Enabled]>"
  In/1 -> Bus Selector Disable Signals/1
  [ASMBUS_ElectricalSystem_Plant] -> ASMSignalInterface/1(ASMSignalBus)

== system ASM_Traffic_new/Engine/Control ==
  note: Engine Basic Control
  Interface_In : Inport
  Plant : Inport  Port=2
  SoftECU_Engine : Subsystem
  UserInterface : Subsystem
  Control : Outport  VectorParamsAs1DForOutWhenUnconnected=off
  wires:
  SoftECU_Engine/1(ASMSignalBus) -> UserInterface/1(In)
  UserInterface/1(Out) -> SoftECU_Engine/1(UserInterface)
  Plant/1 -> SoftECU_Engine/3(Plant)
  SoftECU_Engine/2(Out) -> Control/1
  Interface_In/1 -> SoftECU_Engine/2(Interface_In)

== system ASM_Traffic_new/Engine/Interface_In ==
  note: Engine Basic
  In : Inport
  Bus Creator : BusCreator  Inputs=1
  Bus Selector2 : BusSelector  OutputSignals=Environment.Plant.Sw_ModelPortBlocks[0Disabled|1Enabled],Environment.Plant.Sw_ModelDeskPlottingInterface[0Disabled|1Enabled],DomainControl.TorqueManager.Control.Ignition_ICE[0Off|1On],DomainControl.TorqueManager.Control.StarterReq_ICE[0Off|1On],Drivetrain.Control.Factor_Trq_Engine_Red[%],VehicleDynamics.Control.Enable_TrqDecrease_Fast_ESP[0|1],VehicleDynamics.Control.Trq_DecreaseRequest_Fast_ESP[Nm],VehicleDynamics.Control.Enable_TrqIncrease_ESP[0|1],VehicleDynamics.Control.Trq_IncreaseRequest_ESP[Nm],VehicleDynamics.Control.Enable_TrqDecrease_Slow_ESP[0|1],VehicleDynamics.Control.Trq_DecreaseRequest_Slow_ESP[Nm],DomainControl.TorqueManager.Control.Trq_Request_ICE[Nm],Driver.Plant.Pos_AccPedal[%],Environment.Plant.Reset_States[0|1],Drivetrain.Plant.n_Engine[rpm],Environment.Plant.State_StartButton[-1PowerOff|0Acc|1PowerOn|2StarterOn],DomainControl.TorqueManager.Control.Vehicle_Topology[-2|-1|0|2],VehicleDynamics.Plant.v_x_Vehicle_CoG[km|h],Drivetrain.Plant.Sw_CrankShaft_Reset[0Disabled|1Enabled],Environment.Plant.Mode_StartButtonState[1Stim|2SoftECU],DomainControl.DriverAssistance.Control.Enable_Trq_Increase_ACC[0|1],DomainControl.DriverAssistance.Control.Trq_IncreaseRequest_ACC[Nm]
  Enable_n_Engine_Idle_Request[0|1] : Constant  Value=0
  ModelSignals : Subsystem
  n_Engine_Idle_Request[rpm] : Constant  Value=0
  Out : Outport  VectorParamsAs1DForOutWhenUnconnected=off
  wires:
  Bus Selector2/2 -> ModelSignals/2(Sw_ModelDeskPlottingInterface[0Disabled|1Enabled])  "<Sw_ModelDeskPlottingInterface[0Disabled|1Enabled]>"
  Bus Selector2/1 -> ModelSignals/1(Sw_ModelPortBlocks[0Disabled|1Enabled])  "<Sw_ModelPortBlocks[0Disabled|1Enabled]>"
  In/1 -> Bus Selector2/1
  Bus Selector2/12 -> ModelSignals/12(Trq_Request_ICE[Nm])  "<Trq_Request_ICE[Nm]>"
  Bus Selector2/22 -> ModelSignals/22(Trq_Request_Extern2[Nm])  "<Trq_IncreaseRequest_ACC[Nm]>"
  Bus Selector2/21 -> ModelSignals/21(Enable_Trq_Request_Extern2[0|1])  "<Enable_Trq_Increase_ACC[0|1]>"
  Bus Selector2/7 -> ModelSignals/7(Trq_Decrease_Request_Fast_ESP[Nm])  "<Trq_DecreaseRequest_Fast_ESP[Nm]>"
  Bus Selector2/6 -> ModelSignals/6(Enable_Trq_Decrease_Fast_ESP[0|1])  "<Enable_TrqDecrease_Fast_ESP[0|1]>"
  Bus Selector2/5 -> ModelSignals/5(Factor_Trq_Engine_Red[%])  "<Factor_Trq_Engine_Red[%]>"
  Bus Selector2/4 -> ModelSignals/4(Sw_StarterReq[0Off|1On])  "<StarterReq_ICE[0Off|1On]>"
  Bus Selector2/3 -> ModelSignals/3(Sw_Ignition[0Off|1On])  "<Ignition_ICE[0Off|1On]>"
  Bus Selector2/11 -> ModelSignals/11(Trq_Request_Extern1[Nm])  "<Trq_DecreaseRequest_Slow_ESP[Nm]>"
  Bus Selector2/10 -> ModelSignals/10(Enable_Trq_Request_Extern1[0|1])  "<Enable_TrqDecrease_Slow_ESP[0|1]>"
  Bus Selector2/9 -> ModelSignals/9(Trq_Increase_Request_Fast_ESP[Nm])  "<Trq_IncreaseRequest_ESP[Nm]>"
  Bus Selector2/8 -> ModelSignals/8(Enable_Trq_Increase_Fast_ESP[0|1])  "<Enable_TrqIncrease_ESP[0|1]>"
  Bus Creator/1 -> Out/1
  Enable_n_Engine_Idle_Request[0|1]/1 -> ModelSignals/23(Enable_n_Engine_Idle_Request[0|1])
  n_Engine_Idle_Request[rpm]/1 -> ModelSignals/24(n_Engine_Idle_Request[rpm])
  Bus Selector2/13 -> ModelSignals/13(Pos_AccPedal_Driver[%])  "<Pos_AccPedal[%]>"
  Bus Selector2/14 -> ModelSignals/14(Reset_States[0|1])  "<Reset_States[0|1]>"
  Bus Selector2/15 -> ModelSignals/15(n_Engine[rpm])  "<n_Engine[rpm]>"
  Bus Selector2/16 -> ModelSignals/16(State_StartButton[-1|0|1|2])  "<State_StartButton[-1PowerOff|0Acc|1PowerOn|2StarterOn]>"
  Bus Selector2/17 -> ModelSignals/17(Vehicle_Topology[-2|-1|0|2])  "<Vehicle_Topology[-2|-1|0|2]>"
  Bus Selector2/18 -> ModelSignals/18(v_x_Vehicle[km|h])  "<v_x_Vehicle_CoG[km|h]>"
  Bus Selector2/19 -> ModelSignals/19(Sw_CrankShaft_Reset[0Disabled|1Enabled])  "<Sw_CrankShaft_Reset[0Disabled|1Enabled]>"
  Bus Selector2/20 -> ModelSignals/20(Mode_StartButtonState[1Stim|2SoftECU])  "<Mode_StartButtonState[1Stim|2SoftECU]>"
  ModelSignals/1(Out) -> Bus Creator/1

== system ASM_Traffic_new/Engine/Interface_Out ==
  note: Engine Basic
  In : Inport
  Bus Creator2 : BusCreator  Inputs=2
  Bus Selector2 : BusSelector  OutputSignals=Plant.Engine.Trq_Eff_Engine[Nm],Plant.Engine.Trq_Fric_Engine[Nm]
  Bus Selector6 : BusSelector  OutputSignals=Control.State_Engine[0|1|2|3|4],Control.n_Engine_Idle_Set[rpm],Control.Sw_Starter[0Off|1On],Control.Enable_Trq_Shift_Request[0|1],Control.Trq_Shift_Request[Nm]
  Control_ModelSignals : Subsystem
  CrankAngle_Cyl[aTDC] : Constant  Value=0
  EngOP_Num[] : Constant  Value=0
  Plant_ModelSignals : Subsystem
  Pos_AccPedal_Meas[%] : Constant  Value=0
  State_StartStop[1Off|2NotReady|3Ready|4EngStopped] : Constant
  Sw_Replace_Env[0|1] : Constant  Value=0
  T_Ambient[degC] : Constant  Value=23
  T_Coolant_ICE[degC] : Constant  Value=85
  Trq_MeanEff_Engine_Meas[Nm] : Constant  Value=0
  Type_Engine[0Unkown|1Other|2Otto|3Diesel|4Electric] : Constant
  n_Engine_Meas[rpm] : Constant  Value=0
  p_Ambient[Pa] : Constant  Value=1e5
  Out : Outport  VectorParamsAs1DForOutWhenUnconnected=off
  wires:
  CrankAngle_Cyl[aTDC]/1 -> Control_ModelSignals/7(CrankAngle_Cyl[aTDC])
  T_Ambient[degC]/1 -> Control_ModelSignals/9(T_Ambient[degC])
  p_Ambient[Pa]/1 -> Control_ModelSignals/8(p_Ambient[Pa])
  Trq_MeanEff_Engine_Meas[Nm]/1 -> Control_ModelSignals/14(Trq_MeanEff_Engine_Meas[Nm])
  n_Engine_Meas[rpm]/1 -> Control_ModelSignals/13(n_Engine_Meas[rpm])
  Pos_AccPedal_Meas[%]/1 -> Control_ModelSignals/12(Pos_AccPedal_Meas[%])
  EngOP_Num[]/1 -> Control_ModelSignals/11(EngOP_Num[])
  Sw_Replace_Env[0|1]/1 -> Control_ModelSignals/10(Sw_Replace_Env[0|1])
  Bus Selector6/2 -> Control_ModelSignals/2(n_Engine_Idle_Set[rpm])  "<n_Engine_Idle_Set[rpm]>"
  Bus Selector6/1 -> Control_ModelSignals/1(State_ICEngine[0|1|2|3|4])  "<State_Engine[0|1|2|3|4]>"
  State_StartStop[1Off|2NotReady|3Ready|4EngStopped]/1 -> Control_ModelSignals/6(State_StartStop[1Off|2NotReady|3Ready|4EngStopped])
  T_Coolant_ICE[degC]/1 -> Plant_ModelSignals/3(T_Coolant_ICE[degC])
  Bus Selector2/2 -> Plant_ModelSignals/2(Trq_Fric_Engine[Nm])  "<Trq_Fric_Engine[Nm]>"
  In/1 -> Bus Selector6/1, Bus Selector2/1
  Bus Selector2/1 -> Plant_ModelSignals/1(Trq_MeanEff_Engine[Nm])  "<Trq_Eff_Engine[Nm]>"
  Bus Creator2/1 -> Out/1  "Engine"
  Bus Selector6/3 -> Control_ModelSignals/3(Sw_Starter[0Off|1On])  "<Sw_Starter[0Off|1On]>"
  Bus Selector6/4 -> Control_ModelSignals/4(Enable_Trq_Shift_Request[0|1])  "<Enable_Trq_Shift_Request[0|1]>"
  Bus Selector6/5 -> Control_ModelSignals/5(Trq_Shift_Request[Nm])  "<Trq_Shift_Request[Nm]>"
  Control_ModelSignals/1(Out) -> Bus Creator2/1
  Plant_ModelSignals/1(Out) -> Bus Creator2/2
  Type_Engine[0Unkown|1Other|2Otto|3Diesel|4Electric]/1 -> Plant_ModelSignals/4(Type_Engine[0Unkown|1Other|2Otto|3Diesel|4Electric])

== system ASM_Traffic_new/Engine/Plant ==
  note: Engine Basic
  Interface_In : Inport
  Control : Inport  Port=2
  EngineBasic : Subsystem
  UserInterface : Subsystem
  Plant : Outport  VectorParamsAs1DForOutWhenUnconnected=off
  wires:
  Control/1 -> EngineBasic/3(Control)
  UserInterface/1(Out) -> EngineBasic/1(UserInterface)
  Interface_In/1 -> UserInterface/2(Interface_In), EngineBasic/2(Interface_In)
  EngineBasic/1(ASMSignalBus) -> Plant/1, UserInterface/1(In)

== system ASM_Traffic_new/Engine/SignalInterface ==
  In : Inport
  ASMSignalInterface : Subsystem  mask(ASM_SIGNAL_INTERFACE){LabelTextfield=Engine}
      mask prompts: LabelTextfield "Label"
      mask help:
      | The ASMSignalInterface block processes the ASMSignalBus and provides a vector-based interface for each signal (e.g. ModelDesk Plotting).
      |
      | Always push the update button after you have changed the signal bus structure in order to synchronize the signal interface. The update may take a few seconds.
      | A modified model must be reloaded in ModelDesk to keep consistency of ModelDesk and simulation model plot signals. Therefore select ''Update Model'' from the ''Simulation Model'' context menu of the ModelDesk Project Navigator.
      settings: AttributesFormatString=Label: %<LabelTextfield>
      settings: CopyFcn=|
      | try
      |  set_param(gcb,'LinkStatus', 'none')
      | catch
      | end
      mask Help: eval(['asm_modelhelp(gcbh,''tool'',''ASM_Utils_lib'', ''ASMSIGNALINTERFACE'')'])
      mask DialogControl Hint Prompt: For changes of Label first apply change and then push "Update".
      mask DialogControl UpdateButton Prompt: Update
      mask DialogControl UpdateButton Callback: asm_mdld_plot_block_update(bdroot(gcb), 'update', 'current');
      mask DialogControl UpdateAllButton Prompt: Update All
      mask DialogControl UpdateAllButton Callback: asm_mdld_plot_block_update(bdroot(gcb), 'update', 'all');
  Bus Creator : BusCreator  Inputs=2
  Bus Selector Disable Signals : BusSelector  OutputSignals=ExternalModel.Sw_ModelPortBlocks[0Disabled|1Enabled],ExternalModel.Sw_ModelDeskPlottingInterface[0Disabled|1Enabled]
  ExternalOutports : Subsystem  TreatAsAtomicUnit=on
  wires:
  Bus Selector Disable Signals/2 -> ASMSignalInterface/Enable  "<Sw_ModelDeskPlottingInterface[0Disabled|1Enabled]>"
  Bus Selector Disable Signals/1 -> ExternalOutports/Enable  "<Sw_ModelPortBlocks[0Disabled|1Enabled]>"
  In/1 -> Bus Selector Disable Signals/1
  Bus Creator/1 -> ASMSignalInterface/1(ASMSignalBus), ExternalOutports/1(In1)
  [ASMBUS_Engine_Control] -> Bus Creator/1
  [ASMBUS_Engine_Plant] -> Bus Creator/2

== system ASM_Traffic_new/Environment/GroundTruth ==
  note: GroundTruth
  In : Inport
  Bus Creator2 : BusCreator  Inputs=1
  PlantModel : Subsystem
  UserInterface : Subsystem
  Out : Outport  VectorParamsAs1DForOutWhenUnconnected=off
  wires:
  UserInterface/1(Out) -> PlantModel/1(UserInterface)
  In/1 -> PlantModel/2(In), UserInterface/1(Interface_In)
  PlantModel/1(ASMSignalBus) -> UserInterface/2(In), Bus Creator2/1
  Bus Creator2/1 -> Out/1  "GroundTruth"
